simulink subsystem "tDMSquared_Info"  (R2024b)
settings: Solver=VariableStepAuto  StartTime=0.0  StopTime=10.0  RelTol=1e-3
model mask{messageText='This is a tDMSquared message.', T_s=1e-4}
  mask prompts: messageText "Message Text:"; T_s "Sample Time [s]:"
settings Model: Creator=winkens  LastModifiedBy=k.kocaogullar
settings SolverCC: AlgebraicLoopSolver=TrustRegion
settings OptimizationCC: ReuseModelBlockBuffer=off
settings DebuggingCC: UnconnectedInputMsg=warning  UnconnectedOutputMsg=warning  UnconnectedLineMsg=warning
settings ModelReferenceCC: EnableRefExpFcnMdlSchedulingChecks=on
settings RTWCC: GPUComputeCapability=3.5  DLArmComputeVersion=19.05

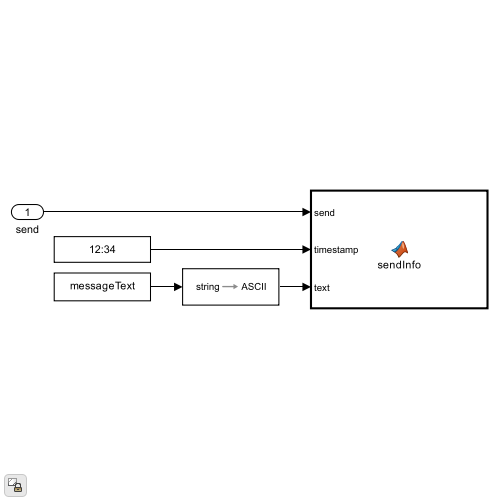
[thumbnail: Simulink's stored preview of the top-level diagram]
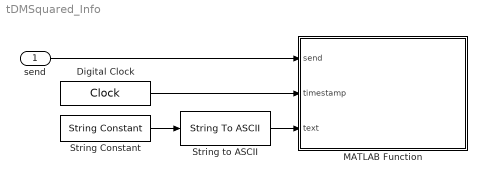
== system tDMSquared_Info ==
  send : Inport
  Digital Clock : DigitalClock  SampleTime=T_s
  MATLAB Function : MATLAB Function  TreatAsAtomicUnit=on
  String Constant : StringConstant  String=messageText  OutDataTypeStr=stringtype(300)
  String to ASCII : StringToASCII  OutputVectorSize=300
  wires:
  send/1 -> MATLAB Function/1(send)
  String Constant/1 -> String to ASCII/1
  Digital Clock/1 -> MATLAB Function/2(timestamp)
  String to ASCII/1 -> MATLAB Function/3(text)

== matlab function tDMSquared_Info/MATLAB Function ==
  data: send input; timestamp input; text input
function sendInfo(send,timestamp, text)
   coder.extrinsic('sldiagviewer.reportInfo');
   coder.extrinsic('gcb');
   %Usage of feval necessary to force usage of Matlab interpreter
   coder.extrinsic('feval');
   if send  
       blockName = gcb;
       message = feval('create_tdm2_Message','info',timestamp,blockName,text);
       sldiagviewer.reportInfo(message);
    end
end
